simulink library "ParameterManager"  (R2025b)
settings: Solver=ode45  StartTime=0.0  StopTime=10.0  RelTol=1e-3  EnableMultiTasking=on
PreLoadFcn:
  | % Please do not Clear this line:
  | %damos=1;
undefined symbols (not defined in the file or in its folder): AD_DrvM_tSTATEIDX_E, u2, u3
libraries: CalibrationLib x21, simulink x10, $bdroot x2
settings Model: Creator=gaz2si  LastModifiedBy=JVE2ST
settings Model: ModifiedHistory=|
  | v7 15.10.2018
  | -Bus Signals removed
  | 
  | v6 07.03.2018
  | 
  | idq current swich in mot param 500us is changed, because of review. No functional changes, only layout.
  | 
  | v5 12.02.2018
  | 
  | Proc Ecu 500us is cahnged because of unit test. One More layer is added.
  | No Functional Changes.
  | 
  | ######################################################################
  | Model Version v4 - 17.08.2017 - ZYU8SI:
  | --------------------------------------------------------------------------------------
  | Developed for SW-Version: 320320_D0101
  | Used in customer projects: Plattform
  | Restrictions:
  | ---------------------------------------------------------------------------------------
  | Changed Interfaces:  - add I/O-Interfaces: fFamosReqd
  | --------------------------------------------------------------------------------------
  | Description:
  | - terminate ComWrp_Outp_iMaxChrgCurrent because no signal available from CAN
  | - set ComWrp_Outp_iChrgCurrDemand(maxDcCurrentOffset)=0. Variable needed for FAMOS
  | 
  | ######################################################################
  | Model Version v3 - 22.02.2017 - ZYU8SI:
  | --------------------------------------------------------------------------------------
  | Developed for SW-Version: latest
  | Used in customer projects: Daimler
  | Restrictions:
  | ---------------------------------------------------------------------------------------
  | Changed Interfaces:  none
  | --------------------------------------------------------------------------------------
  | Description:
  | - Split up model and included all functions as library
  | - from now on no functional development in this lib anymore
  | 
  | ######################################################################
  | 
  | 
  | SOO6SI v2 BMW Version:
  | - Interfaces IdcMin and IdcMax, ResBatteryCharge, ResBatteryDischarge are removed from the ComWrapper,
  |  and replaced by Damos Constants in the mask of the ECUParameter_5ms
  | 
  | ZSD2SI v1 BMW Version:
  | - Interfaces added: CustStMgr_OutP_sState_read
  | - Tq Gradient based on CustStMgr_OutP_sState_read (Torque Gradient has to be positive and in model it has to be set negative aus input)
  | - XCP value considered for Rising and falling Gradient
  | - ParameterManager/ProcEcu_500us/uPhaC_Srv_GetStrtNxtOutpWin set datatype from CSUINT32 to uint32
  | - Multiplikation of coefficients psi_d and psi_q with factor 10^-7
settings SolverCC: AlgebraicLoopSolver=TrustRegion
settings DataIOCC: LimitDataPoints=on  SaveFormat=Array  ReturnWorkspaceOutputs=off
settings OptimizationCC: LifeSpan=inf
settings DebuggingCC: SolverPrmCheckMsg=warning  UnconnectedInputMsg=warning  UnconnectedOutputMsg=warning  UnconnectedLineMsg=warning  AllowSymbolicDim=off  SFUnexpectedBacktrackingDiag=warning  SFNoUnconditionalDefaultTransitionDiag=warning  SFExecutionAtInitializationDiag=none  ArithmeticOperatorsInVariantConditions=warning
settings HardwareCC: ProdBitPerPointer=32.0  ProdBitPerSizeT=32.0  ProdBitPerPtrDiffT=32.0  ProdLargestAtomicFloat=None  ProdIntDivRoundTo=Undefined  ProdEndianess=Unspecified  ProdWordSize=32.0  ProdHWDeviceType=32-bit Generic
settings ModelReferenceCC: EnableRefExpFcnMdlSchedulingChecks=on  PropagateSignalLabelsOutOfModel=off
settings SFSimCC: SimUseLocalCustomCode=off  CustomCodeUndefinedFunction=UseInterfaceOnly
settings RTWCC: RTWUseLocalCustomCode=off  GPUComputeCapability=3.5
settings CodeAppCC: StateflowObjectComments=on
settings GRTTargetCC: TargetLangStandard=C89/C90 (ANSI)
settings ConfigComp: CovMetricSettings=dw  CovSaveCumulativeToWorkspaceVar=on  CovSaveSingleToWorkspaceVar=on  CovExternalEMLEnable=off  CovSFcnEnable=off

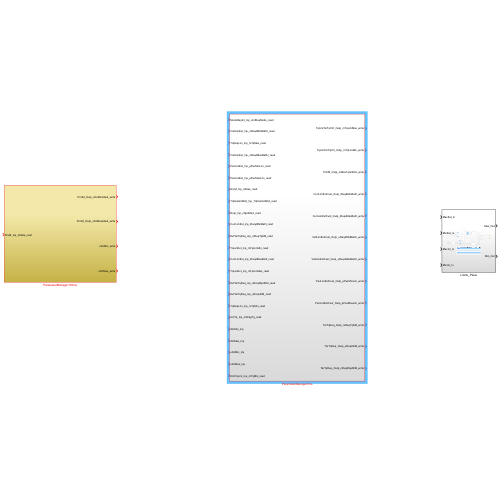
[thumbnail: Simulink's stored preview of the top-level diagram]
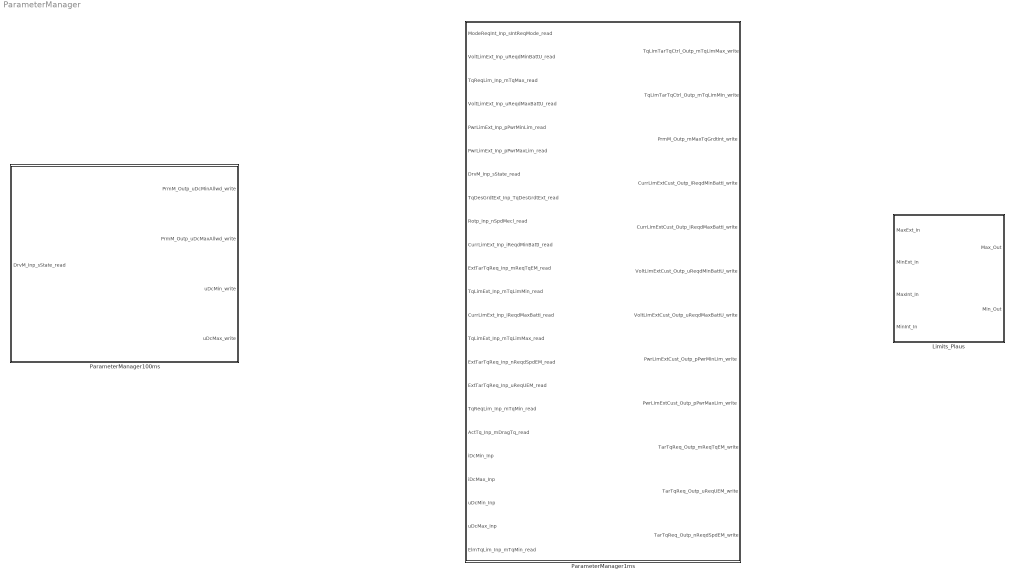
== system ParameterManager ==
  Limits_Plaus : Subsystem
  ParameterManager100ms : Subsystem
  ParameterManager1ms : Subsystem

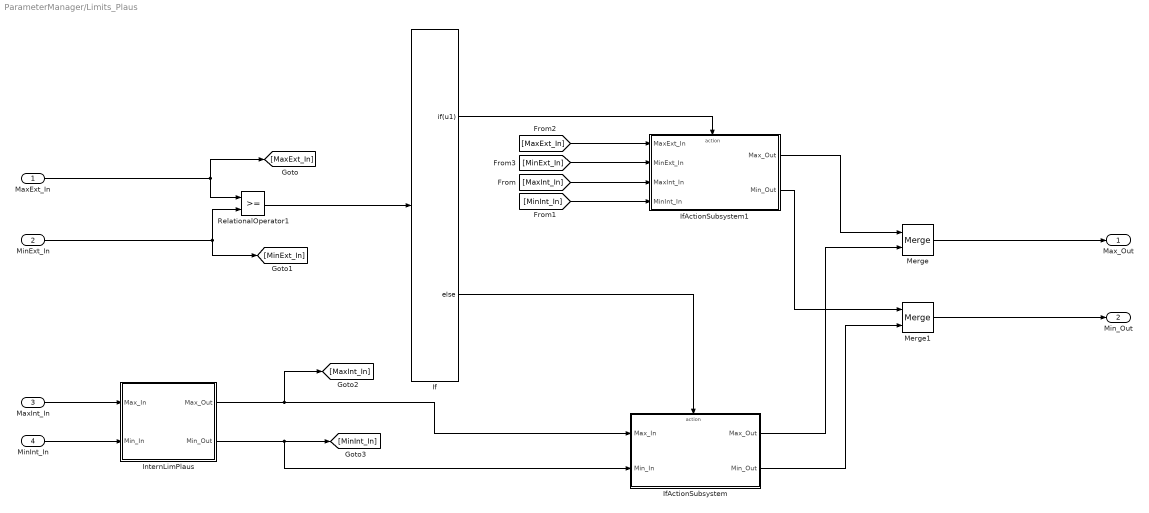
== system ParameterManager/Limits_Plaus ==
  MaxExt_In : Inport
  MinExt_In : Inport  Port=2
  MaxInt_In : Inport  Port=3
  MinInt_In : Inport  Port=4
  If : If  IfExpression=u1
  IfActionSubsystem : Subsystem  TreatAsAtomicUnit=on
  IfActionSubsystem1 : Subsystem  TreatAsAtomicUnit=on
  InternLimPlaus : Subsystem
  Merge : Merge
  Merge1 : Merge
  RelationalOperator1 : RelationalOperator  OutDataTypeStr=boolean  RndMeth=Simplest  InputSameDT=off
  Max_Out : Outport  VectorParamsAs1DForOutWhenUnconnected=off
  Min_Out : Outport  Port=2  VectorParamsAs1DForOutWhenUnconnected=off
  wires:
  If/1 -> IfActionSubsystem1/Action
  RelationalOperator1/1 -> If/1
  MinExt_In/1 -> [MinExt_In], RelationalOperator1/2
  MaxExt_In/1 -> [MaxExt_In], RelationalOperator1/1
  [MinInt_In] -> IfActionSubsystem1/4(MinInt_In)
  InternLimPlaus/2(Min_Out) -> IfActionSubsystem/2(Min_In), [MinInt_In]
  [MaxInt_In] -> IfActionSubsystem1/3(MaxInt_In)
  Merge/1 -> Max_Out/1
  [MaxExt_In] -> IfActionSubsystem1/1(MaxExt_In)
  [MinExt_In] -> IfActionSubsystem1/2(MinExt_In)
  If/2 -> IfActionSubsystem/Action
  InternLimPlaus/1(Max_Out) -> [MaxInt_In], IfActionSubsystem/1(Max_In)
  IfActionSubsystem1/2(Min_Out) -> Merge1/1
  IfActionSubsystem/1(Max_Out) -> Merge/2
  IfActionSubsystem1/1(Max_Out) -> Merge/1
  Merge1/1 -> Min_Out/1
  IfActionSubsystem/2(Min_Out) -> Merge1/2
  MaxInt_In/1 -> InternLimPlaus/1(Max_In)
  MinInt_In/1 -> InternLimPlaus/2(Min_In)

== system ParameterManager/ParameterManager100ms ==
  DrvM_Inp_sState_read : Inport
  ElectricalLimits : Subsystem
  SendingParameters : Subsystem
  PrmM_Outp_uDcMinAllwd_write : Outport  OutDataTypeStr=single  VectorParamsAs1DForOutWhenUnconnected=off
  PrmM_Outp_uDcMaxAllwd_write : Outport  Port=2  OutDataTypeStr=single  VectorParamsAs1DForOutWhenUnconnected=off
  uDcMin_write : Outport  Port=3  OutMin=24  OutMax=54  OutDataTypeStr=AD_PrmM_tUDCMINALLWD  PortDimensions=1  VectorParamsAs1DForOutWhenUnconnected=off
  uDcMax_write : Outport  Port=4  OutMin=24  OutMax=54  OutDataTypeStr=AD_PrmM_tUDCMAXALLWD  PortDimensions=1  VectorParamsAs1DForOutWhenUnconnected=off
  wires:
  DrvM_Inp_sState_read/1 -> ElectricalLimits/1(sState)
  ElectricalLimits/1(uDcMin_write) -> SendingParameters/1(uDcMin), uDcMin_write/1
  ElectricalLimits/2(uDcMax_write) -> SendingParameters/2(uDcMax), uDcMax_write/1
  SendingParameters/1(uDcMin_write) -> PrmM_Outp_uDcMinAllwd_write/1
  SendingParameters/2(uDcMax_write) -> PrmM_Outp_uDcMaxAllwd_write/1

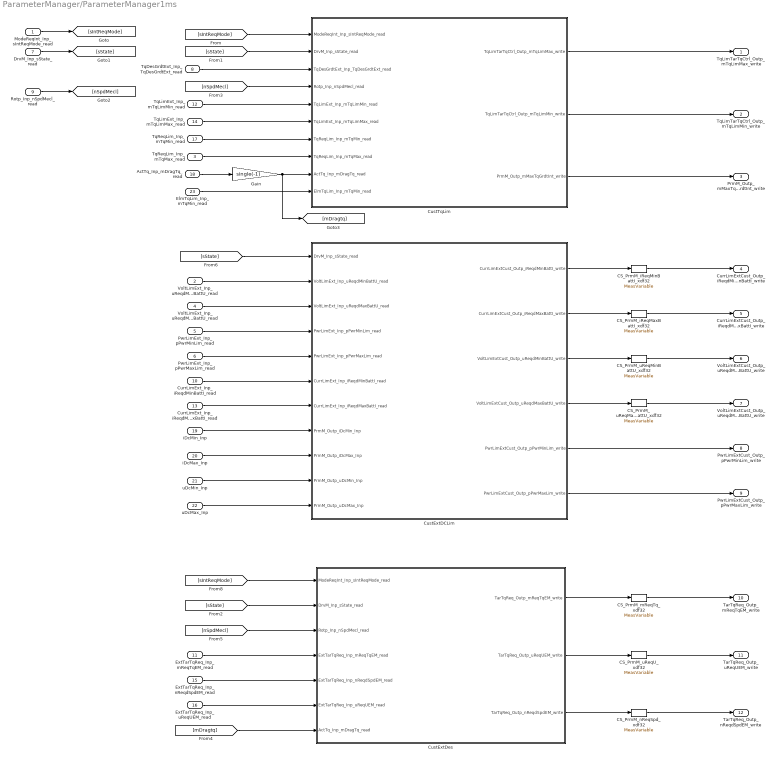
== system ParameterManager/ParameterManager1ms ==
  ModeReqInt_Inp_sIntReqMode_read : Inport
  VoltLimExt_Inp_uReqdMinBattU_read : Inport  Port=2
  TqReqLim_Inp_mTqMax_read : Inport  Port=3
  VoltLimExt_Inp_uReqdMaxBattU_read : Inport  Port=4
  PwrLimExt_Inp_pPwrMinLim_read : Inport  Port=5
  PwrLimExt_Inp_pPwrMaxLim_read : Inport  Port=6
  DrvM_Inp_sState_read : Inport  Port=7
  TqDesGrdtExt_Inp_TqDesGrdtExt_read : Inport  Port=8
  Rotp_Inp_nSpdMecl_read : Inport  Port=9
  CurrLimExt_Inp_iReqdMinBattI_read : Inport  Port=10
  ExtTarTqReq_Inp_mReqTqEM_read : Inport  Port=11
  TqLimExt_Inp_mTqLimMin_read : Inport  Port=12
  CurrLimExt_Inp_iReqdMaxBattI_read : Inport  Port=13
  TqLimExt_Inp_mTqLimMax_read : Inport  Port=14
  ExtTarTqReq_Inp_nReqdSpdEM_read : Inport  Port=15
  ExtTarTqReq_Inp_uReqUEM_read : Inport  Port=16
  TqReqLim_Inp_mTqMin_read : Inport  Port=17
  ActTq_Inp_mDragTq_read : Inport  Port=18
  iDcMin_Inp : Inport  Port=19
  iDcMax_Inp : Inport  Port=20
  uDcMin_Inp : Inport  Port=21
  uDcMax_Inp : Inport  Port=22
  ElmTqLim_Inp_mTqMin_read : Inport  Port=23
  CS_PrmM_iReqMaxBattI_xdf32 : CalibrationLib/MeasVariable  calSigName=CS_PrmM_iReqMaxBattI_xdf32  logSignal=on
      settings: AttributesFormatString=%<calSigName>  SourceProductName=SEG Calibration Lib
  CS_PrmM_iReqMinBattI_xdf32 : CalibrationLib/MeasVariable  calSigName=CS_PrmM_iReqMinBattI_xdf32  logSignal=on
      settings: AttributesFormatString=%<calSigName>  SourceProductName=SEG Calibration Lib
  CS_PrmM_mReqTq_xdf32 : CalibrationLib/MeasVariable  calSigName=CS_PrmM_mReqTq_xdf32  logSignal=on
      settings: AttributesFormatString=%<calSigName>  SourceProductName=SEG Calibration Lib
  CS_PrmM_nReqSpd_xdf32 : CalibrationLib/MeasVariable  calSigName=CS_PrmM_nReqSpd_xdf32  logSignal=on
      settings: AttributesFormatString=%<calSigName>  SourceProductName=SEG Calibration Lib
  CS_PrmM_uReqMaxBattU_xdf32 : CalibrationLib/MeasVariable  calSigName=CS_PrmM_uReqMaxBattU_xdf32  logSignal=on
      settings: AttributesFormatString=%<calSigName>  SourceProductName=SEG Calibration Lib
  CS_PrmM_uReqMinBattU_xdf32 : CalibrationLib/MeasVariable  calSigName=CS_PrmM_uReqMinBattU_xdf32  logSignal=on
      settings: AttributesFormatString=%<calSigName>  SourceProductName=SEG Calibration Lib
  CS_PrmM_uReqU_xdf32 : CalibrationLib/MeasVariable  calSigName=CS_PrmM_uReqU_xdf32  logSignal=on
      settings: AttributesFormatString=%<calSigName>  SourceProductName=SEG Calibration Lib
  CustExtDCLim : Subsystem
  CustExtDes : Subsystem
  CustTqLim : Subsystem
  Gain : Gain  Gain=single(-1)
  TqLimTarTqCtrl_Outp_mTqLimMax_write : Outport  VectorParamsAs1DForOutWhenUnconnected=off
      settings: EnsureOutportIsVirtual=on
  TqLimTarTqCtrl_Outp_mTqLimMin_write : Outport  Port=2  VectorParamsAs1DForOutWhenUnconnected=off
      settings: EnsureOutportIsVirtual=on
  PrmM_Outp_mMaxTqGrdtInt_write : Outport  Port=3  VectorParamsAs1DForOutWhenUnconnected=off
      settings: EnsureOutportIsVirtual=on
  CurrLimExtCust_Outp_iReqdMinBattI_write : Outport  Port=4  VectorParamsAs1DForOutWhenUnconnected=off
      settings: EnsureOutportIsVirtual=on
  CurrLimExtCust_Outp_iReqdMaxBattI_write : Outport  Port=5  VectorParamsAs1DForOutWhenUnconnected=off
      settings: EnsureOutportIsVirtual=on
  VoltLimExtCust_Outp_uReqdMinBattU_write : Outport  Port=6  VectorParamsAs1DForOutWhenUnconnected=off
      settings: EnsureOutportIsVirtual=on
  VoltLimExtCust_Outp_uReqdMaxBattU_write : Outport  Port=7  VectorParamsAs1DForOutWhenUnconnected=off
      settings: EnsureOutportIsVirtual=on
  PwrLimExtCust_Outp_pPwrMinLim_write : Outport  Port=8  VectorParamsAs1DForOutWhenUnconnected=off
      settings: EnsureOutportIsVirtual=on
  PwrLimExtCust_Outp_pPwrMaxLim_write : Outport  Port=9  VectorParamsAs1DForOutWhenUnconnected=off
      settings: EnsureOutportIsVirtual=on
  TarTqReq_Outp_mReqTqEM_write : Outport  Port=10  VectorParamsAs1DForOutWhenUnconnected=off
      settings: EnsureOutportIsVirtual=on
  TarTqReq_Outp_uReqUEM_write : Outport  Port=11  VectorParamsAs1DForOutWhenUnconnected=off
      settings: EnsureOutportIsVirtual=on
  TarTqReq_Outp_nReqdSpdEM_write : Outport  Port=12  VectorParamsAs1DForOutWhenUnconnected=off
      settings: EnsureOutportIsVirtual=on
  wires:
  Gain/1 -> [mDragtq], CustTqLim/9(ActTq_Inp_mDragTq_read)
  [mDragtq] -> CustExtDes/7(ActTq_Inp_mDragTq_read)
  ElmTqLim_Inp_mTqMin_read/1 -> CustTqLim/10(ElmTqLim_Inp_mTqMin_read)
  TqReqLim_Inp_mTqMax_read/1 -> CustTqLim/8(TqReqLim_Inp_mTqMax_read)
  VoltLimExt_Inp_uReqdMaxBattU_read/1 -> CustExtDCLim/3(VoltLimExt_Inp_uReqdMaxBattU_read)
  PwrLimExt_Inp_pPwrMinLim_read/1 -> CustExtDCLim/4(PwrLimExt_Inp_pPwrMinLim_read)
  PwrLimExt_Inp_pPwrMaxLim_read/1 -> CustExtDCLim/5(PwrLimExt_Inp_pPwrMaxLim_read)
  DrvM_Inp_sState_read/1 -> [sState]
  TqDesGrdtExt_Inp_TqDesGrdtExt_read/1 -> CustTqLim/3(TqDesGrdtExt_Inp_TqDesGrdtExt_read)
  Rotp_Inp_nSpdMecl_read/1 -> [nSpdMecl]
  CurrLimExt_Inp_iReqdMinBattI_read/1 -> CustExtDCLim/6(CurrLimExt_Inp_iReqdMinBattI_read)
  ExtTarTqReq_Inp_mReqTqEM_read/1 -> CustExtDes/4(ExtTarTqReq_Inp_mReqTqEM_read)
  TqLimExt_Inp_mTqLimMin_read/1 -> CustTqLim/5(TqLimExt_Inp_mTqLimMin_read)
  CurrLimExt_Inp_iReqdMaxBattI_read/1 -> CustExtDCLim/7(CurrLimExt_Inp_iReqdMaxBattI_read)
  TqLimExt_Inp_mTqLimMax_read/1 -> CustTqLim/6(TqLimExt_Inp_mTqLimMax_read)
  ExtTarTqReq_Inp_nReqdSpdEM_read/1 -> CustExtDes/5(ExtTarTqReq_Inp_nReqdSpdEM_read)
  ExtTarTqReq_Inp_uReqUEM_read/1 -> CustExtDes/6(ExtTarTqReq_Inp_uReqUEM_read)
  ActTq_Inp_mDragTq_read/1 -> Gain/1
  CustExtDCLim/1(CurrLimExtCust_Outp_iReqdMinBattI_write) -> CS_PrmM_iReqMinBattI_xdf32/1
  CustExtDCLim/2(CurrLimExtCust_Outp_iReqdMaxBattI_write) -> CS_PrmM_iReqMaxBattI_xdf32/1
  CustExtDCLim/3(VoltLimExtCust_Outp_uReqdMinBattU_write) -> CS_PrmM_uReqMinBattU_xdf32/1
  CustExtDCLim/4(VoltLimExtCust_Outp_uReqdMaxBattU_write) -> CS_PrmM_uReqMaxBattU_xdf32/1
  CustExtDCLim/5(PwrLimExtCust_Outp_pPwrMinLim_write) -> PwrLimExtCust_Outp_pPwrMinLim_write/1
  CustExtDCLim/6(PwrLimExtCust_Outp_pPwrMaxLim_write) -> PwrLimExtCust_Outp_pPwrMaxLim_write/1
  CustExtDes/1(TarTqReq_Outp_mReqTqEM_write) -> CS_PrmM_mReqTq_xdf32/1
  CustExtDes/2(TarTqReq_Outp_uReqUEM_write) -> CS_PrmM_uReqU_xdf32/1
  CustExtDes/3(TarTqReq_Outp_nReqdSpdEM_write) -> CS_PrmM_nReqSpd_xdf32/1
  iDcMin_Inp/1 -> CustExtDCLim/8(PrmM_Outp_iDcMin_Inp)
  iDcMax_Inp/1 -> CustExtDCLim/9(PrmM_Outp_iDcMax_Inp)
  uDcMin_Inp/1 -> CustExtDCLim/10(PrmM_Outp_uDcMin_Inp)
  uDcMax_Inp/1 -> CustExtDCLim/11(PrmM_Outp_uDcMax_Inp)
  ModeReqInt_Inp_sIntReqMode_read/1 -> [sIntReqMode]
  [sIntReqMode] -> CustTqLim/1(ModeReqInt_Inp_sIntReqMode_read)
  [sIntReqMode] -> CustExtDes/1(ModeReqInt_Inp_sIntReqMode_read)
  [sState] -> CustTqLim/2(DrvM_Inp_sState_read)
  [sState] -> CustExtDes/2(DrvM_Inp_sState_read)
  TqReqLim_Inp_mTqMin_read/1 -> CustTqLim/7(TqReqLim_Inp_mTqMin_read)
  [nSpdMecl] -> CustTqLim/4(Rotp_Inp_nSpdMecl_read)
  VoltLimExt_Inp_uReqdMinBattU_read/1 -> CustExtDCLim/2(VoltLimExt_Inp_uReqdMinBattU_read)
  [nSpdMecl] -> CustExtDes/3(Rotp_Inp_nSpdMecl_read)
  CustTqLim/1(TqLimTarTqCtrl_Outp_mTqLimMax_write) -> TqLimTarTqCtrl_Outp_mTqLimMax_write/1
  CustTqLim/2(TqLimTarTqCtrl_Outp_mTqLimMin_write) -> TqLimTarTqCtrl_Outp_mTqLimMin_write/1
  CS_PrmM_iReqMinBattI_xdf32/1 -> CurrLimExtCust_Outp_iReqdMinBattI_write/1
  CS_PrmM_iReqMaxBattI_xdf32/1 -> CurrLimExtCust_Outp_iReqdMaxBattI_write/1
  CS_PrmM_uReqMinBattU_xdf32/1 -> VoltLimExtCust_Outp_uReqdMinBattU_write/1
  CS_PrmM_mReqTq_xdf32/1 -> TarTqReq_Outp_mReqTqEM_write/1
  CS_PrmM_uReqU_xdf32/1 -> TarTqReq_Outp_uReqUEM_write/1
  CS_PrmM_nReqSpd_xdf32/1 -> TarTqReq_Outp_nReqdSpdEM_write/1
  CS_PrmM_uReqMaxBattU_xdf32/1 -> VoltLimExtCust_Outp_uReqdMaxBattU_write/1
  CustTqLim/3(PrmM_Outp_mMaxTqGrdtInt_write) -> PrmM_Outp_mMaxTqGrdtInt_write/1
  [sState] -> CustExtDCLim/1(DrvM_Inp_sState_read)

== system ParameterManager/Limits_Plaus/IfActionSubsystem ==
  Max_In : Inport
  Min_In : Inport  Port=2
  ActionPort : ActionPort
  Max_Out : Outport  VectorParamsAs1DForOutWhenUnconnected=off
  Min_Out : Outport  Port=2  VectorParamsAs1DForOutWhenUnconnected=off
  wires:
  Max_In/1 -> Max_Out/1
  Min_In/1 -> Min_Out/1

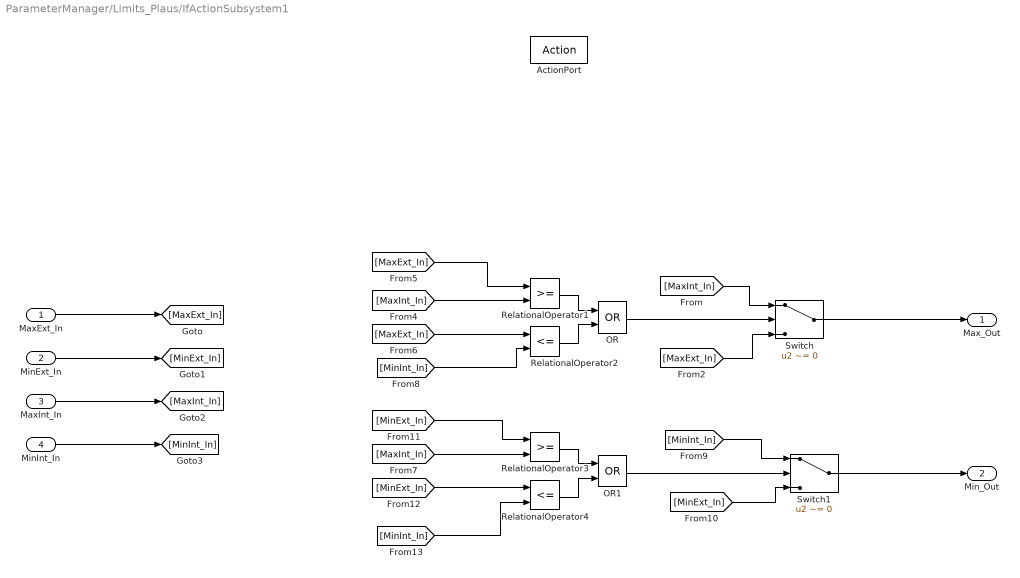
== system ParameterManager/Limits_Plaus/IfActionSubsystem1 ==
  MaxExt_In : Inport
  MinExt_In : Inport  Port=2
  MaxInt_In : Inport  Port=3
  MinInt_In : Inport  Port=4
  ActionPort : ActionPort  ActionPortLabel=if { }
  OR : Logic  Operator=OR  AllPortsSameDT=off  OutDataTypeStr=boolean
  OR1 : Logic  Operator=OR  AllPortsSameDT=off  OutDataTypeStr=boolean
  RelationalOperator1 : RelationalOperator  OutDataTypeStr=boolean  RndMeth=Simplest  InputSameDT=off
  RelationalOperator2 : RelationalOperator  Operator=<=  OutDataTypeStr=boolean  RndMeth=Simplest  InputSameDT=off
  RelationalOperator3 : RelationalOperator  OutDataTypeStr=boolean  RndMeth=Simplest  InputSameDT=off
  RelationalOperator4 : RelationalOperator  Operator=<=  OutDataTypeStr=boolean  RndMeth=Simplest  InputSameDT=off
  Switch : Switch  Criteria=u2 ~= 0  SaturateOnIntegerOverflow=off  InputSameDT=off
  Switch1 : Switch  Criteria=u2 ~= 0  SaturateOnIntegerOverflow=off  InputSameDT=off
  Max_Out : Outport  VectorParamsAs1DForOutWhenUnconnected=off
  Min_Out : Outport  Port=2  VectorParamsAs1DForOutWhenUnconnected=off
  wires:
  Switch1/1 -> Min_Out/1
  Switch/1 -> Max_Out/1
  MaxExt_In/1 -> [MaxExt_In]
  MaxInt_In/1 -> [MaxInt_In]
  MinInt_In/1 -> [MinInt_In]
  RelationalOperator1/1 -> OR/1
  RelationalOperator2/1 -> OR/2
  OR/1 -> Switch/2
  RelationalOperator4/1 -> OR1/2
  RelationalOperator3/1 -> OR1/1
  OR1/1 -> Switch1/2
  MinExt_In/1 -> [MinExt_In]
  [MaxExt_In] -> Switch/3
  [MaxInt_In] -> Switch/1
  [MaxInt_In] -> RelationalOperator1/2
  [MaxExt_In] -> RelationalOperator1/1
  [MaxExt_In] -> RelationalOperator2/1
  [MaxInt_In] -> RelationalOperator3/2
  [MinInt_In] -> RelationalOperator2/2
  [MinInt_In] -> Switch1/1
  [MinExt_In] -> Switch1/3
  [MinExt_In] -> RelationalOperator3/1
  [MinExt_In] -> RelationalOperator4/1
  [MinInt_In] -> RelationalOperator4/2

== system ParameterManager/Limits_Plaus/InternLimPlaus ==
  Max_In : Inport
  Min_In : Inport  Port=2
  RelationalOperator1 : RelationalOperator  OutDataTypeStr=boolean  RndMeth=Simplest  InputSameDT=off
  Switch : Switch  Criteria=u2 ~= 0  SaturateOnIntegerOverflow=off  InputSameDT=off
  Switch1 : Switch  Criteria=u2 ~= 0  SaturateOnIntegerOverflow=off  InputSameDT=off
  Max_Out : Outport  VectorParamsAs1DForOutWhenUnconnected=off
  Min_Out : Outport  Port=2  VectorParamsAs1DForOutWhenUnconnected=off
  wires:
  RelationalOperator1/1 -> Switch1/2, Switch/2
  Max_In/1 -> Switch1/3, Switch/1, RelationalOperator1/1
  Switch/1 -> Max_Out/1
  Switch1/1 -> Min_Out/1
  Min_In/1 -> RelationalOperator1/2, Switch/3, Switch1/1

== system ParameterManager/ParameterManager100ms/ElectricalLimits ==
  sState : Inport
  BatterylessOperation : Subsystem  TreatAsAtomicUnit=on
  CompareToConstant : simulink/Logic and Bit Operations/Compare To Constant  relop===  const=AD_DrvM_tSTATEIDX_E.CS_DrvM_STATE_BattDiscnctd  OutDataTypeStr=boolean
  CompareToConstant1 : simulink/Logic and Bit Operations/Compare To Constant  relop===  const=AD_DrvM_tSTATEIDX_E.CS_DrvM_STATE_Volt  OutDataTypeStr=boolean
  If : If  NumInputs=2  IfExpression=u1  ElseIfExpressions=u2
  Merge : Merge  Inputs=3
  Merge1 : Merge  Inputs=3
  Other : Subsystem  TreatAsAtomicUnit=on
  VoltageMode : Subsystem  TreatAsAtomicUnit=on
  uDcMin_write : Outport  OutMin=20  OutMax=65  OutDataTypeStr=AD_PrmM_tUDCMINALLWD  PortDimensions=1  VectorParamsAs1DForOutWhenUnconnected=off
  uDcMax_write : Outport  Port=2  OutMin=20  OutMax=65  OutDataTypeStr=AD_PrmM_tUDCMAXALLWD  PortDimensions=1  VectorParamsAs1DForOutWhenUnconnected=off
  wires:
  Other/1(uUmin) -> Merge/3
  CompareToConstant/1 -> If/1
  VoltageMode/2(uUmax) -> Merge1/2
  CompareToConstant1/1 -> If/2
  If/1 -> BatterylessOperation/Action
  sState/1 -> CompareToConstant1/1, CompareToConstant/1
  Merge1/1 -> uDcMax_write/1
  VoltageMode/1(uUmin) -> Merge/2
  If/2 -> VoltageMode/Action
  If/3 -> Other/Action
  BatterylessOperation/1(uUmin) -> Merge/1
  BatterylessOperation/2(uUmax) -> Merge1/1
  Other/2(uUmax) -> Merge1/3
  Merge/1 -> uDcMin_write/1

== system ParameterManager/ParameterManager100ms/SendingParameters ==
  uDcMin : Inport
  uDcMax : Inport  Port=2
  uDcMin_write : Outport  OutMin=20  OutMax=65  OutDataTypeStr=AD_PrmM_tUDCMINALLWD  PortDimensions=1  VectorParamsAs1DForOutWhenUnconnected=off
  uDcMax_write : Outport  Port=2  OutMin=20  OutMax=65  OutDataTypeStr=AD_PrmM_tUDCMAXALLWD  PortDimensions=1  VectorParamsAs1DForOutWhenUnconnected=off
  wires:
  uDcMin/1 -> uDcMin_write/1
  uDcMax/1 -> uDcMax_write/1

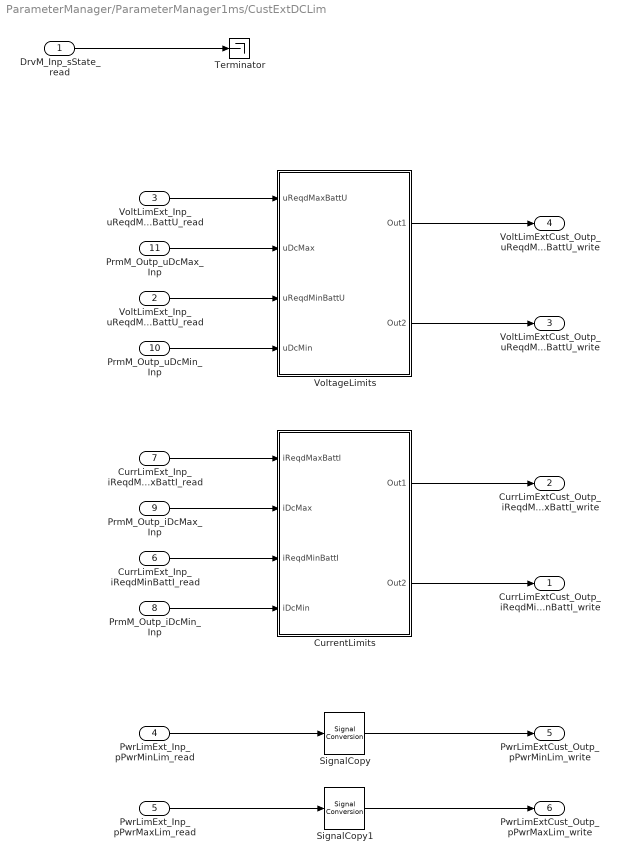
== system ParameterManager/ParameterManager1ms/CustExtDCLim ==
  DrvM_Inp_sState_read : Inport
  VoltLimExt_Inp_uReqdMinBattU_read : Inport  Port=2
  VoltLimExt_Inp_uReqdMaxBattU_read : Inport  Port=3
  PwrLimExt_Inp_pPwrMinLim_read : Inport  Port=4
  PwrLimExt_Inp_pPwrMaxLim_read : Inport  Port=5
  CurrLimExt_Inp_iReqdMinBattI_read : Inport  Port=6
  CurrLimExt_Inp_iReqdMaxBattI_read : Inport  Port=7
  PrmM_Outp_iDcMin_Inp : Inport  Port=8
  PrmM_Outp_iDcMax_Inp : Inport  Port=9
  PrmM_Outp_uDcMin_Inp : Inport  Port=10
  PrmM_Outp_uDcMax_Inp : Inport  Port=11
  CurrentLimits : Subsystem
  SignalCopy : SignalConversion  OverrideOpt=off
  SignalCopy1 : SignalConversion  OverrideOpt=off
  Terminator : Terminator
  VoltageLimits : Subsystem
  CurrLimExtCust_Outp_iReqdMinBattI_write : Outport  VectorParamsAs1DForOutWhenUnconnected=off
      settings: EnsureOutportIsVirtual=on
  CurrLimExtCust_Outp_iReqdMaxBattI_write : Outport  Port=2  VectorParamsAs1DForOutWhenUnconnected=off
      settings: EnsureOutportIsVirtual=on
  VoltLimExtCust_Outp_uReqdMinBattU_write : Outport  Port=3  VectorParamsAs1DForOutWhenUnconnected=off
      settings: EnsureOutportIsVirtual=on
  VoltLimExtCust_Outp_uReqdMaxBattU_write : Outport  Port=4  VectorParamsAs1DForOutWhenUnconnected=off
      settings: EnsureOutportIsVirtual=on
  PwrLimExtCust_Outp_pPwrMinLim_write : Outport  Port=5  VectorParamsAs1DForOutWhenUnconnected=off
      settings: EnsureOutportIsVirtual=on
  PwrLimExtCust_Outp_pPwrMaxLim_write : Outport  Port=6  VectorParamsAs1DForOutWhenUnconnected=off
      settings: EnsureOutportIsVirtual=on
  wires:
  VoltLimExt_Inp_uReqdMaxBattU_read/1 -> VoltageLimits/1(uReqdMaxBattU)
  PrmM_Outp_uDcMax_Inp/1 -> VoltageLimits/2(uDcMax)
  VoltLimExt_Inp_uReqdMinBattU_read/1 -> VoltageLimits/3(uReqdMinBattU)
  PrmM_Outp_uDcMin_Inp/1 -> VoltageLimits/4(uDcMin)
  VoltageLimits/1(Out1) -> VoltLimExtCust_Outp_uReqdMaxBattU_write/1
  VoltageLimits/2(Out2) -> VoltLimExtCust_Outp_uReqdMinBattU_write/1
  CurrentLimits/2(Out2) -> CurrLimExtCust_Outp_iReqdMinBattI_write/1
  CurrentLimits/1(Out1) -> CurrLimExtCust_Outp_iReqdMaxBattI_write/1
  CurrLimExt_Inp_iReqdMaxBattI_read/1 -> CurrentLimits/1(iReqdMaxBattI)
  PrmM_Outp_iDcMax_Inp/1 -> CurrentLimits/2(iDcMax)
  PrmM_Outp_iDcMin_Inp/1 -> CurrentLimits/4(iDcMin)
  CurrLimExt_Inp_iReqdMinBattI_read/1 -> CurrentLimits/3(iReqdMinBattI)
  PwrLimExt_Inp_pPwrMaxLim_read/1 -> SignalCopy1/1
  SignalCopy/1 -> PwrLimExtCust_Outp_pPwrMinLim_write/1
  SignalCopy1/1 -> PwrLimExtCust_Outp_pPwrMaxLim_write/1
  PwrLimExt_Inp_pPwrMinLim_read/1 -> SignalCopy/1
  DrvM_Inp_sState_read/1 -> Terminator/1

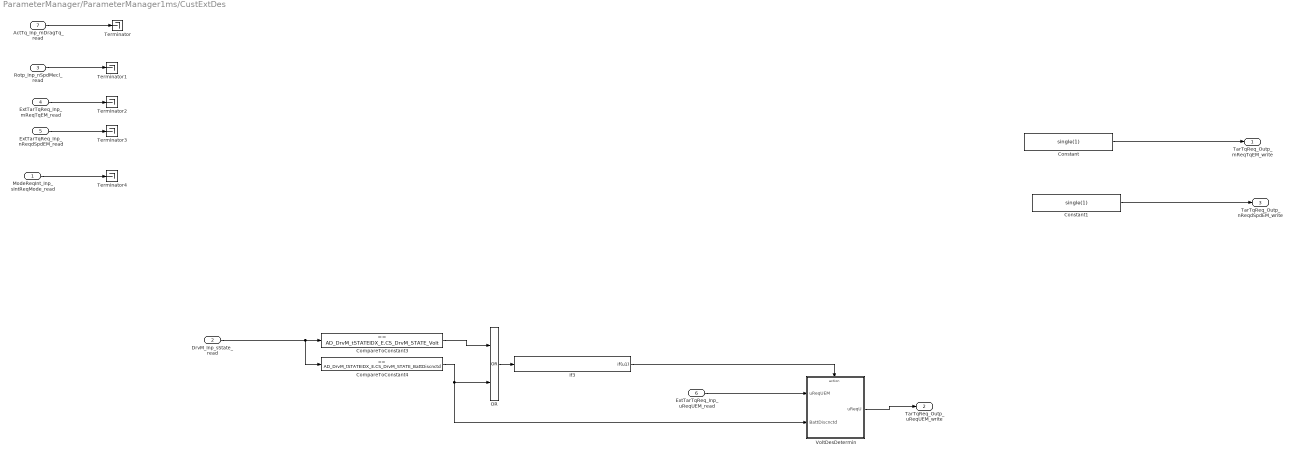
== system ParameterManager/ParameterManager1ms/CustExtDes ==
  ModeReqInt_Inp_sIntReqMode_read : Inport
  DrvM_Inp_sState_read : Inport  Port=2
  Rotp_Inp_nSpdMecl_read : Inport  Port=3
  ExtTarTqReq_Inp_mReqTqEM_read : Inport  Port=4
  ExtTarTqReq_Inp_nReqdSpdEM_read : Inport  Port=5
  ExtTarTqReq_Inp_uReqUEM_read : Inport  Port=6
  ActTq_Inp_mDragTq_read : Inport  Port=7
  CompareToConstant3 : simulink/Logic and Bit Operations/Compare To Constant  relop===  const=AD_DrvM_tSTATEIDX_E.CS_DrvM_STATE_Volt  OutDataTypeStr=boolean
  CompareToConstant4 : simulink/Logic and Bit Operations/Compare To Constant  relop===  const=AD_DrvM_tSTATEIDX_E.CS_DrvM_STATE_BattDiscnctd  OutDataTypeStr=boolean
  Constant : Constant  Value=single(1)
  Constant1 : Constant  Value=single(1)
  If3 : If  IfExpression=u1  ShowElse=off
  OR : Logic  Operator=OR  AllPortsSameDT=off  OutDataTypeStr=boolean
  Terminator{,1..4} (5 alike) : Terminator
  VoltDesDetermin : Subsystem  TreatAsAtomicUnit=on
  TarTqReq_Outp_mReqTqEM_write : Outport  VectorParamsAs1DForOutWhenUnconnected=off
      settings: EnsureOutportIsVirtual=on
  TarTqReq_Outp_uReqUEM_write : Outport  Port=2  VectorParamsAs1DForOutWhenUnconnected=off
      settings: EnsureOutportIsVirtual=on
  TarTqReq_Outp_nReqdSpdEM_write : Outport  Port=3  VectorParamsAs1DForOutWhenUnconnected=off
      settings: EnsureOutportIsVirtual=on
  wires:
  ExtTarTqReq_Inp_uReqUEM_read/1 -> VoltDesDetermin/1(uReqUEM)
  Constant1/1 -> TarTqReq_Outp_nReqdSpdEM_write/1
  DrvM_Inp_sState_read/1 -> CompareToConstant3/1, CompareToConstant4/1
  OR/1 -> If3/1
  CompareToConstant3/1 -> OR/1
  CompareToConstant4/1 -> VoltDesDetermin/2(BattDiscnctd), OR/2
  VoltDesDetermin/1(uReqU) -> TarTqReq_Outp_uReqUEM_write/1
  If3/1 -> VoltDesDetermin/Action
  ActTq_Inp_mDragTq_read/1 -> Terminator/1
  Rotp_Inp_nSpdMecl_read/1 -> Terminator1/1
  ExtTarTqReq_Inp_nReqdSpdEM_read/1 -> Terminator3/1
  ExtTarTqReq_Inp_mReqTqEM_read/1 -> Terminator2/1
  ModeReqInt_Inp_sIntReqMode_read/1 -> Terminator4/1
  Constant/1 -> TarTqReq_Outp_mReqTqEM_write/1

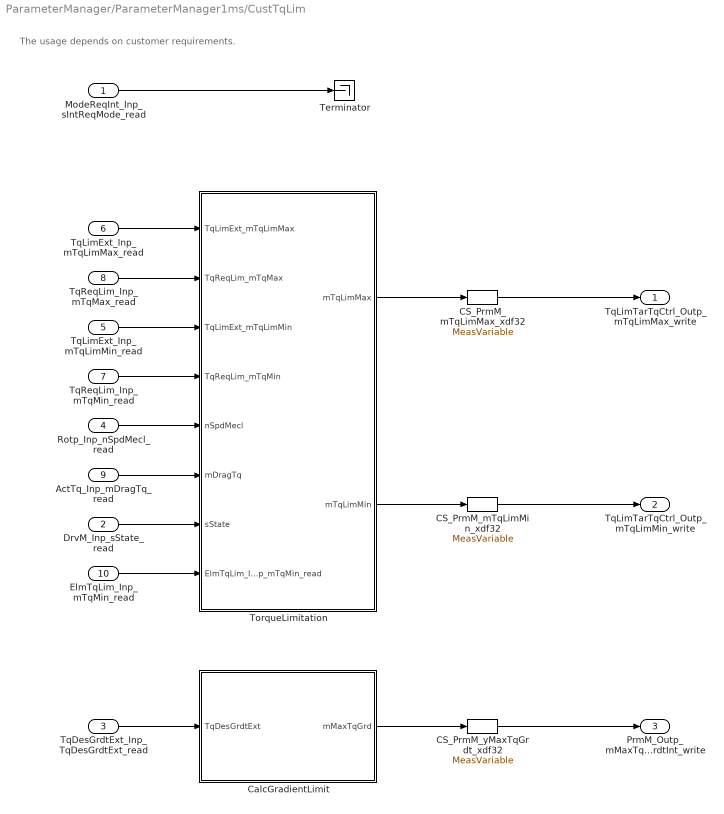
== system ParameterManager/ParameterManager1ms/CustTqLim ==
  note: The usage depends on customer requirements.
  ModeReqInt_Inp_sIntReqMode_read : Inport
  DrvM_Inp_sState_read : Inport  Port=2
  TqDesGrdtExt_Inp_TqDesGrdtExt_read : Inport  Port=3
  Rotp_Inp_nSpdMecl_read : Inport  Port=4
  TqLimExt_Inp_mTqLimMin_read : Inport  Port=5
  TqLimExt_Inp_mTqLimMax_read : Inport  Port=6
  TqReqLim_Inp_mTqMin_read : Inport  Port=7
  TqReqLim_Inp_mTqMax_read : Inport  Port=8
  ActTq_Inp_mDragTq_read : Inport  Port=9
  ElmTqLim_Inp_mTqMin_read : Inport  Port=10
  CS_PrmM_mTqLimMax_xdf32 : CalibrationLib/MeasVariable  calSigName=CS_PrmM_mTqLimMax_xdf32  logSignal=on
      settings: AttributesFormatString=%<calSigName>  SourceProductName=SEG Calibration Lib
  CS_PrmM_mTqLimMin_xdf32 : CalibrationLib/MeasVariable  calSigName=CS_PrmM_mTqLimMin_xdf32  logSignal=on
      settings: AttributesFormatString=%<calSigName>  SourceProductName=SEG Calibration Lib
  CS_PrmM_yMaxTqGrdt_xdf32 : CalibrationLib/MeasVariable  calSigName=CS_PrmM_yMaxTqGrdt_xdf32  logSignal=on
      settings: AttributesFormatString=%<calSigName>  SourceProductName=SEG Calibration Lib
  CalcGradientLimit : Subsystem
  Terminator : Terminator
  TorqueLimitation : Subsystem
  TqLimTarTqCtrl_Outp_mTqLimMax_write : Outport  VectorParamsAs1DForOutWhenUnconnected=off
      settings: EnsureOutportIsVirtual=on
  TqLimTarTqCtrl_Outp_mTqLimMin_write : Outport  Port=2  VectorParamsAs1DForOutWhenUnconnected=off
      settings: EnsureOutportIsVirtual=on
  PrmM_Outp_mMaxTqGrdtInt_write : Outport  Port=3  VectorParamsAs1DForOutWhenUnconnected=off
      settings: EnsureOutportIsVirtual=on
  wires:
  ElmTqLim_Inp_mTqMin_read/1 -> TorqueLimitation/8(ElmTqLim_Inp_mTqMin_read)
  ModeReqInt_Inp_sIntReqMode_read/1 -> Terminator/1
  TorqueLimitation/1(mTqLimMax) -> CS_PrmM_mTqLimMax_xdf32/1
  TqDesGrdtExt_Inp_TqDesGrdtExt_read/1 -> CalcGradientLimit/1(TqDesGrdtExt)
  CalcGradientLimit/1(mMaxTqGrd) -> CS_PrmM_yMaxTqGrdt_xdf32/1
  TqLimExt_Inp_mTqLimMax_read/1 -> TorqueLimitation/1(TqLimExt_mTqLimMax)
  TqReqLim_Inp_mTqMax_read/1 -> TorqueLimitation/2(TqReqLim_mTqMax)
  TqLimExt_Inp_mTqLimMin_read/1 -> TorqueLimitation/3(TqLimExt_mTqLimMin)
  TqReqLim_Inp_mTqMin_read/1 -> TorqueLimitation/4(TqReqLim_mTqMin)
  Rotp_Inp_nSpdMecl_read/1 -> TorqueLimitation/5(nSpdMecl)
  ActTq_Inp_mDragTq_read/1 -> TorqueLimitation/6(mDragTq)
  DrvM_Inp_sState_read/1 -> TorqueLimitation/7(sState)
  TorqueLimitation/2(mTqLimMin) -> CS_PrmM_mTqLimMin_xdf32/1
  CS_PrmM_mTqLimMax_xdf32/1 -> TqLimTarTqCtrl_Outp_mTqLimMax_write/1
  CS_PrmM_mTqLimMin_xdf32/1 -> TqLimTarTqCtrl_Outp_mTqLimMin_write/1
  CS_PrmM_yMaxTqGrdt_xdf32/1 -> PrmM_Outp_mMaxTqGrdtInt_write/1

== system ParameterManager/ParameterManager100ms/ElectricalLimits/BatterylessOperation ==
  ActionPort : ActionPort  ActionPortLabel=if { }
  CS_PrmM_uDcMaxBattLess_XDF32 : CalibrationLib/Parameter  calParamName=CS_PrmM_uDcMaxBattLess_XDF32
      settings: AttributesFormatString=%<calParamName>  SourceProductName=SEG Calibration Lib
  CS_PrmM_uDcMinBattLess_XDF32 : CalibrationLib/Parameter  calParamName=CS_PrmM_uDcMinBattLess_XDF32
      settings: AttributesFormatString=%<calParamName>  SourceProductName=SEG Calibration Lib
  uUmin : Outport  VectorParamsAs1DForOutWhenUnconnected=off
  uUmax : Outport  Port=2  VectorParamsAs1DForOutWhenUnconnected=off
  wires:
  CS_PrmM_uDcMaxBattLess_XDF32/1 -> uUmax/1
  CS_PrmM_uDcMinBattLess_XDF32/1 -> uUmin/1

== system ParameterManager/ParameterManager100ms/ElectricalLimits/Other ==
  ActionPort : ActionPort  ActionPortLabel=else { }
  CS_PrmM_uDcMaxOtherM_XDF32 : CalibrationLib/Parameter  calParamName=CS_PrmM_uDcMaxOtherM_XDF32
      settings: AttributesFormatString=%<calParamName>  SourceProductName=SEG Calibration Lib
  CS_PrmM_uDcMinOtherM_XDF32 : CalibrationLib/Parameter  calParamName=CS_PrmM_uDcMinOtherM_XDF32
      settings: AttributesFormatString=%<calParamName>  SourceProductName=SEG Calibration Lib
  uUmin : Outport  VectorParamsAs1DForOutWhenUnconnected=off
  uUmax : Outport  Port=2  VectorParamsAs1DForOutWhenUnconnected=off
  wires:
  CS_PrmM_uDcMinOtherM_XDF32/1 -> uUmin/1
  CS_PrmM_uDcMaxOtherM_XDF32/1 -> uUmax/1

== system ParameterManager/ParameterManager100ms/ElectricalLimits/VoltageMode ==
  ActionPort : ActionPort  ActionPortLabel=elseif { }
  CS_PrmM_uDcMaxVoltMode_XDF32 : CalibrationLib/Parameter  calParamName=CS_PrmM_uDcMaxVoltMode_XDF32
      settings: AttributesFormatString=%<calParamName>  SourceProductName=SEG Calibration Lib
  CS_PrmM_uDcMinVoltMode_XDF32 : CalibrationLib/Parameter  calParamName=CS_PrmM_uDcMinVoltMode_XDF32
      settings: AttributesFormatString=%<calParamName>  SourceProductName=SEG Calibration Lib
  uUmin : Outport  VectorParamsAs1DForOutWhenUnconnected=off
  uUmax : Outport  Port=2  VectorParamsAs1DForOutWhenUnconnected=off
  wires:
  CS_PrmM_uDcMaxVoltMode_XDF32/1 -> uUmax/1
  CS_PrmM_uDcMinVoltMode_XDF32/1 -> uUmin/1

== system ParameterManager/ParameterManager1ms/CustExtDCLim/CurrentLimits ==
  iReqdMaxBattI : Inport
  iDcMax : Inport  Port=2
  iReqdMinBattI : Inport  Port=3
  iDcMin : Inport  Port=4
  Limits_Plaus : $bdroot/Limits_Plaus  SystemSampleTime=-1  VariantActivationTime=update diagram  EmptyChoice=off  PassThrough=off  PassThroughVariantControl=(default)  EmptyChoiceVariantControl=(default)  AllowFlexibleInterface=on  Latency=0  AutoFrameSizeCalculation=off
  Out1 : Outport  VectorParamsAs1DForOutWhenUnconnected=off
  Out2 : Outport  Port=2  VectorParamsAs1DForOutWhenUnconnected=off
  wires:
  Limits_Plaus/1 -> Out1/1
  Limits_Plaus/2 -> Out2/1
  iReqdMaxBattI/1 -> Limits_Plaus/1
  iDcMax/1 -> Limits_Plaus/3
  iReqdMinBattI/1 -> Limits_Plaus/2
  iDcMin/1 -> Limits_Plaus/4

== system ParameterManager/ParameterManager1ms/CustExtDCLim/VoltageLimits ==
  uReqdMaxBattU : Inport
  uDcMax : Inport  Port=2
  uReqdMinBattU : Inport  Port=3
  uDcMin : Inport  Port=4
  Limits_Plaus : $bdroot/Limits_Plaus  SystemSampleTime=-1  VariantActivationTime=update diagram  EmptyChoice=off  PassThrough=off  PassThroughVariantControl=(default)  EmptyChoiceVariantControl=(default)  AllowFlexibleInterface=on  Latency=0  AutoFrameSizeCalculation=off
  Out1 : Outport  VectorParamsAs1DForOutWhenUnconnected=off
  Out2 : Outport  Port=2  VectorParamsAs1DForOutWhenUnconnected=off
  wires:
  Limits_Plaus/2 -> Out2/1
  Limits_Plaus/1 -> Out1/1
  uReqdMaxBattU/1 -> Limits_Plaus/1
  uReqdMinBattU/1 -> Limits_Plaus/2
  uDcMax/1 -> Limits_Plaus/3
  uDcMin/1 -> Limits_Plaus/4

== system ParameterManager/ParameterManager1ms/CustExtDes/VoltDesDetermin ==
  uReqUEM : Inport
  BattDiscnctd : Inport  Port=2
  ActionPort : ActionPort
  Saturation : Saturate  UpperLimit=single(54.5)  LowerLimit=single(24)
      settings: AttributesFormatString=|
      | UpperLim: %<UpperLimit>
      | LowerLim: %<LowerLimit>
  Switch1 : Switch  Criteria=u2 ~= 0  SaturateOnIntegerOverflow=off  InputSameDT=off
  uReqU : Outport  VectorParamsAs1DForOutWhenUnconnected=off
  wires:
  Switch1/1 -> uReqU/1
  BattDiscnctd/1 -> Switch1/2
  Saturation/1 -> Switch1/1
  uReqUEM/1 -> Switch1/3, Saturation/1

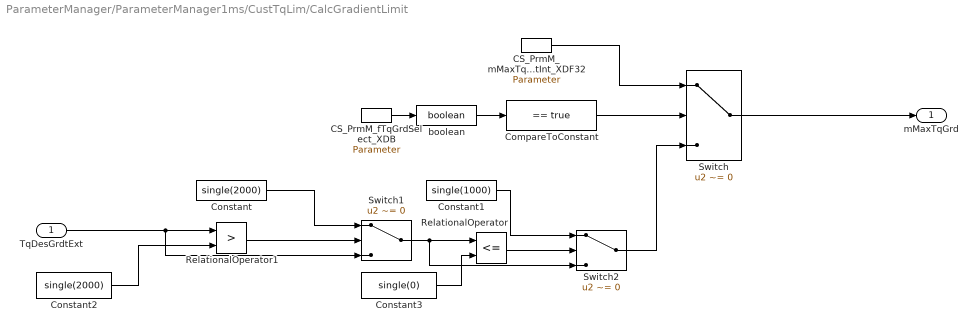
== system ParameterManager/ParameterManager1ms/CustTqLim/CalcGradientLimit ==
  TqDesGrdtExt : Inport
  CS_PrmM_fTqGrdSelect_XDB : CalibrationLib/Parameter  calParamName=CS_PrmM_fTqGrdSelect_XDB
      settings: AttributesFormatString=%<calParamName>  SourceProductName=SEG Calibration Lib
  CS_PrmM_mMaxTqGrdtInt_XDF32 : CalibrationLib/Parameter  calParamName=CS_PrmM_mMaxTqGrdtInt_XDF32
      settings: AttributesFormatString=%<calParamName>  SourceProductName=SEG Calibration Lib
  CompareToConstant : simulink/Logic and Bit Operations/Compare To Constant  relop===  const=true  OutDataTypeStr=boolean
  Constant : Constant  Value=single(2000)
  Constant1 : Constant  Value=single(1000)
  Constant2 : Constant  Value=single(2000)
  Constant3 : Constant  Value=single(0)
  RelationalOperator : RelationalOperator  Operator=<=  OutDataTypeStr=boolean  RndMeth=Simplest  InputSameDT=off
  RelationalOperator1 : RelationalOperator  Operator=>  OutDataTypeStr=boolean  RndMeth=Simplest  InputSameDT=off
  Switch : Switch  Criteria=u2 ~= 0  SaturateOnIntegerOverflow=off  InputSameDT=off
  Switch1 : Switch  Criteria=u2 ~= 0  SaturateOnIntegerOverflow=off  InputSameDT=off
  Switch2 : Switch  Criteria=u2 ~= 0  SaturateOnIntegerOverflow=off  InputSameDT=off
  boolean : DataTypeConversion  OutDataTypeStr=boolean  SaturateOnIntegerOverflow=off  RndMeth=Floor
  mMaxTqGrd : Outport  VectorParamsAs1DForOutWhenUnconnected=off
  wires:
  RelationalOperator/1 -> Switch2/2
  Constant/1 -> Switch1/1
  Constant1/1 -> Switch2/1
  TqDesGrdtExt/1 -> Switch1/3, RelationalOperator1/1
  Switch/1 -> mMaxTqGrd/1
  Switch2/1 -> Switch/3
  RelationalOperator1/1 -> Switch1/2
  Switch1/1 -> RelationalOperator/1, Switch2/3
  CS_PrmM_mMaxTqGrdtInt_XDF32/1 -> Switch/1
  Constant2/1 -> RelationalOperator1/2
  Constant3/1 -> RelationalOperator/2
  CS_PrmM_fTqGrdSelect_XDB/1 -> boolean/1
  boolean/1 -> CompareToConstant/1
  CompareToConstant/1 -> Switch/2

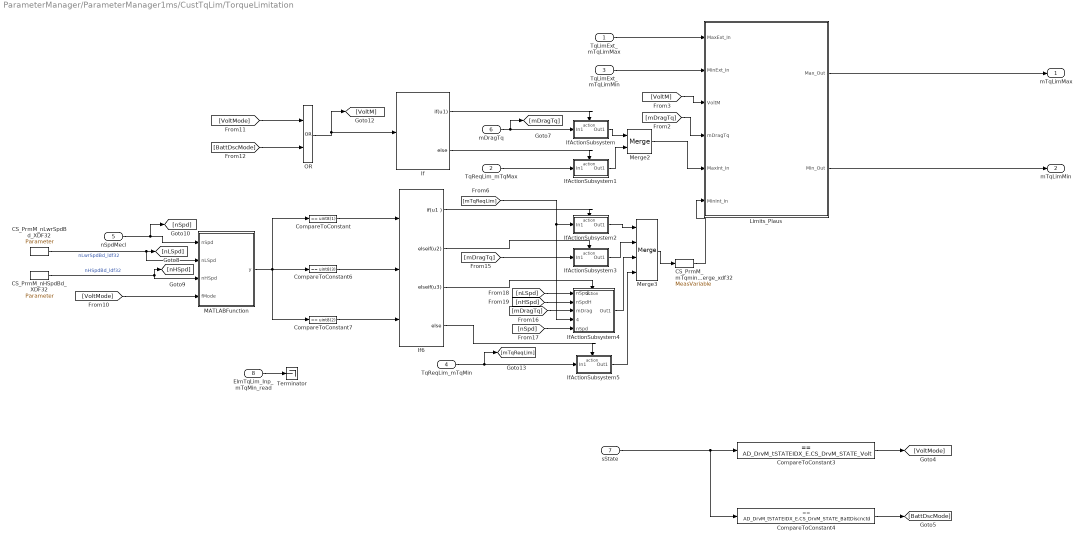
== system ParameterManager/ParameterManager1ms/CustTqLim/TorqueLimitation ==
  TqLimExt_mTqLimMax : Inport
  TqReqLim_mTqMax : Inport  Port=2
  TqLimExt_mTqLimMin : Inport  Port=3
  TqReqLim_mTqMin : Inport  Port=4
  nSpdMecl : Inport  Port=5
  mDragTq : Inport  Port=6
  sState : Inport  Port=7
  ElmTqLim_Inp_mTqMin_read : Inport  Port=8
  CS_PrmM_mTqminmerge_xdf32 : CalibrationLib/MeasVariable  calSigName=CS_PrmM_mTqminmerge_xdf32  logSignal=on
      settings: AttributesFormatString=%<calSigName>  SourceProductName=SEG Calibration Lib
  CS_PrmM_nHSpdBd_XDF32 : CalibrationLib/Parameter  calParamName=CS_PrmM_nHSpdBd_XDF32
      settings: AttributesFormatString=%<calParamName>  SourceProductName=SEG Calibration Lib
  CS_PrmM_nLwrSpdBd_XDF32 : CalibrationLib/Parameter  calParamName=CS_PrmM_nLwrSpdBd_XDF32
      settings: AttributesFormatString=%<calParamName>  SourceProductName=SEG Calibration Lib
  CompareToConstant : simulink/Logic and Bit Operations/Compare To Constant  relop===  const=uint8(1)  OutDataTypeStr=boolean
  CompareToConstant3 : simulink/Logic and Bit Operations/Compare To Constant  relop===  const=AD_DrvM_tSTATEIDX_E.CS_DrvM_STATE_Volt  OutDataTypeStr=boolean
  CompareToConstant4 : simulink/Logic and Bit Operations/Compare To Constant  relop===  const=AD_DrvM_tSTATEIDX_E.CS_DrvM_STATE_BattDiscnctd  OutDataTypeStr=boolean
  CompareToConstant6 : simulink/Logic and Bit Operations/Compare To Constant  relop===  const=uint8(3)  OutDataTypeStr=boolean
  CompareToConstant7 : simulink/Logic and Bit Operations/Compare To Constant  relop===  const=uint8(2)  OutDataTypeStr=boolean
  If : If  IfExpression=u1
  If6 : If  NumInputs=3  IfExpression=u1  ElseIfExpressions=u2,u3
  IfActionSubsystem : Subsystem  TreatAsAtomicUnit=on
  IfActionSubsystem1 : Subsystem  TreatAsAtomicUnit=on
  IfActionSubsystem2 : Subsystem  TreatAsAtomicUnit=on
  IfActionSubsystem3 : Subsystem  TreatAsAtomicUnit=on
  IfActionSubsystem4 : Subsystem  TreatAsAtomicUnit=on
  IfActionSubsystem5 : Subsystem  TreatAsAtomicUnit=on
  Limits_Plaus : Subsystem  AncestorBlock=ParameterManager/Limits_Plaus
  MATLABFunction : MATLAB Function  TreatAsAtomicUnit=on
  Merge2 : Merge
  Merge3 : Merge  Inputs=4
  OR : Logic  Operator=OR  AllPortsSameDT=off  OutDataTypeStr=boolean
  Terminator : Terminator
  mTqLimMax : Outport  VectorParamsAs1DForOutWhenUnconnected=off
  mTqLimMin : Outport  Port=2  VectorParamsAs1DForOutWhenUnconnected=off
  wires:
  [mDragTq] -> Limits_Plaus/4(mDragTq)
  nSpdMecl/1 -> [nSpd], MATLABFunction/1(nSpd)
  CompareToConstant/1 -> If6/1
  CS_PrmM_nHSpdBd_XDF32/1 -> MATLABFunction/3(nHSpd), [nHSpd]  "nHSpdBd_ldf32"
  CS_PrmM_nLwrSpdBd_XDF32/1 -> MATLABFunction/2(nLSpd), [nLSpd]  "nLwrSpdBd_ldf32"
  Merge2/1 -> Limits_Plaus/5(MaxInt_In)
  IfActionSubsystem1/1(Out1) -> Merge2/2
  TqReqLim_mTqMax/1 -> IfActionSubsystem1/1(In1)
  IfActionSubsystem/1(Out1) -> Merge2/1
  mDragTq/1 -> [mDragTq], IfActionSubsystem/1(In1)
  If/2 -> IfActionSubsystem1/Action
  If/1 -> IfActionSubsystem/Action
  OR/1 -> [VoltM], If/1
  [BattDscMode] -> OR/2
  [VoltMode] -> OR/1
  Limits_Plaus/1(Max_Out) -> mTqLimMax/1
  Limits_Plaus/2(Min_Out) -> mTqLimMin/1
  TqLimExt_mTqLimMin/1 -> Limits_Plaus/2(MinExt_In)
  TqLimExt_mTqLimMax/1 -> Limits_Plaus/1(MaxExt_In)
  sState/1 -> CompareToConstant4/1, CompareToConstant3/1
  [VoltMode] -> MATLABFunction/4(fMode)
  MATLABFunction/1(y) -> CompareToConstant/1, CompareToConstant6/1, CompareToConstant7/1
  If6/1 -> IfActionSubsystem2/Action
  ElmTqLim_Inp_mTqMin_read/1 -> Terminator/1
  IfActionSubsystem2/1(Out1) -> Merge3/1
  CompareToConstant6/1 -> If6/2
  CompareToConstant7/1 -> If6/3
  If6/2 -> IfActionSubsystem3/Action
  [mDragTq] -> IfActionSubsystem3/1(In1)
  IfActionSubsystem3/1(Out1) -> Merge3/2
  If6/3 -> IfActionSubsystem4/Action
  IfActionSubsystem4/1(Out1) -> Merge3/3
  If6/4 -> IfActionSubsystem5/Action
  TqReqLim_mTqMin/1 -> [mTqReqLim], IfActionSubsystem5/1(In1)
  IfActionSubsystem5/1(Out1) -> Merge3/4
  Merge3/1 -> CS_PrmM_mTqminmerge_xdf32/1
  CompareToConstant3/1 -> [VoltMode]
  CompareToConstant4/1 -> [BattDscMode]
  [VoltM] -> Limits_Plaus/3(VoltM)
  CS_PrmM_mTqminmerge_xdf32/1 -> Limits_Plaus/6(MinInt_In)
  [mDragTq] -> IfActionSubsystem4/3(mDrag)
  [nSpd] -> IfActionSubsystem4/5(nSpd)
  [nLSpd] -> IfActionSubsystem4/1(nSpdL)
  [nHSpd] -> IfActionSubsystem4/2(nSpdH)
  [mTqReqLim] -> IfActionSubsystem4/4(mTqMin), IfActionSubsystem2/1(In1)

== system ParameterManager/ParameterManager1ms/CustTqLim/TorqueLimitation/IfActionSubsystem ==
  In1 : Inport
  ActionPort : ActionPort
  Out1 : Outport  VectorParamsAs1DForOutWhenUnconnected=off
  wires:
  In1/1 -> Out1/1

== system ParameterManager/ParameterManager1ms/CustTqLim/TorqueLimitation/IfActionSubsystem1 ==
  In1 : Inport
  ActionPort : ActionPort
  Out1 : Outport  VectorParamsAs1DForOutWhenUnconnected=off
  wires:
  In1/1 -> Out1/1

== system ParameterManager/ParameterManager1ms/CustTqLim/TorqueLimitation/IfActionSubsystem2 ==
  In1 : Inport
  ActionPort : ActionPort
  Out1 : Outport  VectorParamsAs1DForOutWhenUnconnected=off
  wires:
  In1/1 -> Out1/1

== system ParameterManager/ParameterManager1ms/CustTqLim/TorqueLimitation/IfActionSubsystem3 ==
  In1 : Inport
  ActionPort : ActionPort
  Out1 : Outport  VectorParamsAs1DForOutWhenUnconnected=off
  wires:
  In1/1 -> Out1/1

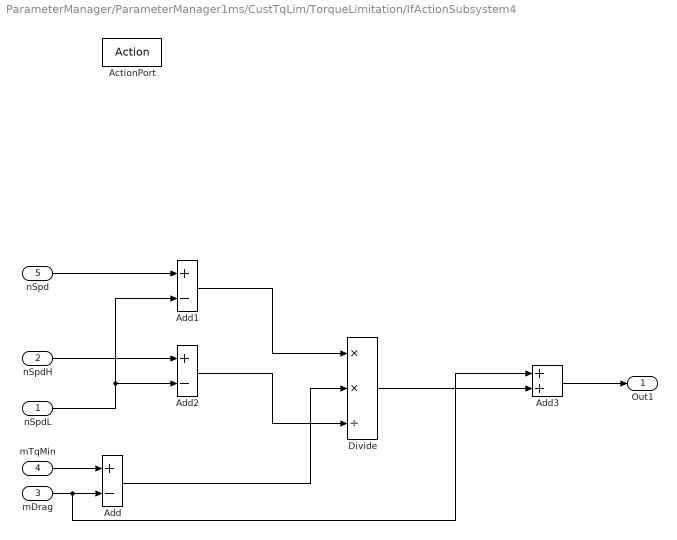
== system ParameterManager/ParameterManager1ms/CustTqLim/TorqueLimitation/IfActionSubsystem4 ==
  nSpdL : Inport
  nSpdH : Inport  Port=2
  mDrag : Inport  Port=3
  mTqMin : Inport  Port=4
  nSpd : Inport  Port=5
  ActionPort : ActionPort
  Add : Sum  Inputs=+-
  Add1 : Sum  Inputs=+-
  Add2 : Sum  Inputs=+-
  Add3 : Sum
  Divide : Product  Inputs=**/
  Out1 : Outport  VectorParamsAs1DForOutWhenUnconnected=off
  wires:
  mTqMin/1 -> Add/1
  mDrag/1 -> Add3/1, Add/2
  nSpd/1 -> Add1/1
  nSpdL/1 -> Add2/2, Add1/2
  nSpdH/1 -> Add2/1
  Add2/1 -> Divide/3
  Add1/1 -> Divide/1
  Add/1 -> Divide/2
  Divide/1 -> Add3/2
  Add3/1 -> Out1/1

== system ParameterManager/ParameterManager1ms/CustTqLim/TorqueLimitation/IfActionSubsystem5 ==
  In1 : Inport
  ActionPort : ActionPort
  Out1 : Outport  VectorParamsAs1DForOutWhenUnconnected=off
  wires:
  In1/1 -> Out1/1

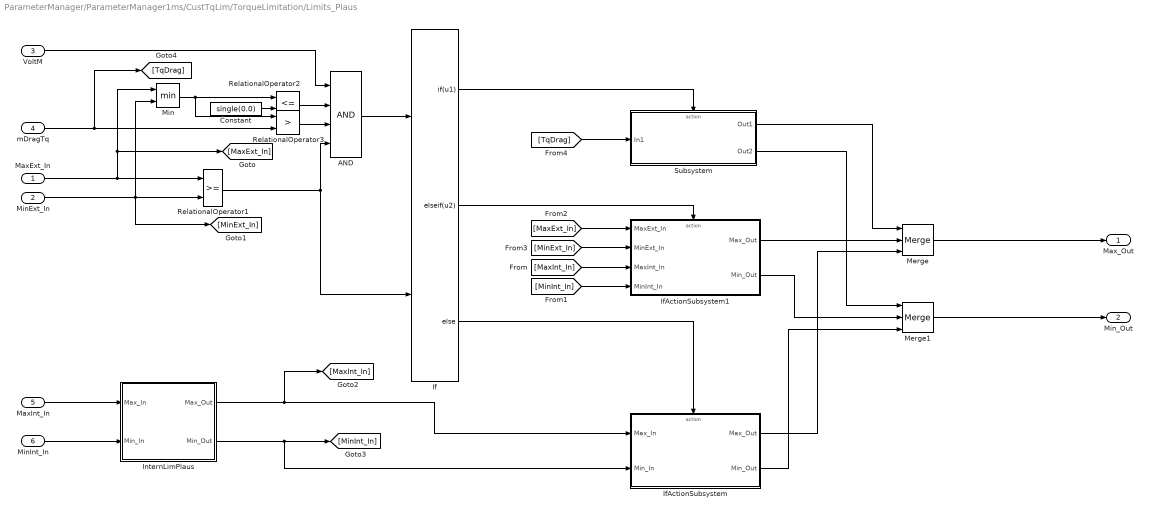
== system ParameterManager/ParameterManager1ms/CustTqLim/TorqueLimitation/Limits_Plaus ==
  MaxExt_In : Inport
  MinExt_In : Inport  Port=2
  VoltM : Inport  Port=3
  mDragTq : Inport  Port=4
  MaxInt_In : Inport  Port=5
  MinInt_In : Inport  Port=6
  AND : Logic  Inputs=4  AllPortsSameDT=off  OutDataTypeStr=boolean
  Constant : Constant  Value=single(0.0)
  If : If  NumInputs=2  IfExpression=u1  ElseIfExpressions=u2
  IfActionSubsystem : Subsystem  TreatAsAtomicUnit=on
  IfActionSubsystem1 : Subsystem  TreatAsAtomicUnit=on
  InternLimPlaus : Subsystem
  Merge : Merge  Inputs=3
  Merge1 : Merge  Inputs=3
  Min : MinMax  Inputs=2
  RelationalOperator1 : RelationalOperator  OutDataTypeStr=boolean  RndMeth=Simplest  InputSameDT=off
  RelationalOperator2 : RelationalOperator  Operator=<=  OutDataTypeStr=boolean  RndMeth=Simplest  InputSameDT=off
  RelationalOperator3 : RelationalOperator  Operator=>  OutDataTypeStr=boolean  RndMeth=Simplest  InputSameDT=off
  Subsystem : Subsystem
  Max_Out : Outport  VectorParamsAs1DForOutWhenUnconnected=off
  Min_Out : Outport  Port=2  VectorParamsAs1DForOutWhenUnconnected=off
  wires:
  MinInt_In/1 -> InternLimPlaus/2(Min_In)
  MaxInt_In/1 -> InternLimPlaus/1(Max_In)
  IfActionSubsystem/2(Min_Out) -> Merge1/3
  Merge1/1 -> Min_Out/1
  IfActionSubsystem1/1(Max_Out) -> Merge/2
  IfActionSubsystem/1(Max_Out) -> Merge/3
  IfActionSubsystem1/2(Min_Out) -> Merge1/2
  InternLimPlaus/1(Max_Out) -> IfActionSubsystem/1(Max_In), [MaxInt_In]
  If/3 -> IfActionSubsystem/Action
  [MinExt_In] -> IfActionSubsystem1/2(MinExt_In)
  [MaxExt_In] -> IfActionSubsystem1/1(MaxExt_In)
  Merge/1 -> Max_Out/1
  [MaxInt_In] -> IfActionSubsystem1/3(MaxInt_In)
  InternLimPlaus/2(Min_Out) -> [MinInt_In], IfActionSubsystem/2(Min_In)
  [MinInt_In] -> IfActionSubsystem1/4(MinInt_In)
  MaxExt_In/1 -> [MaxExt_In], Min/1, RelationalOperator1/1
  MinExt_In/1 -> Min/2, RelationalOperator1/2, [MinExt_In]
  Min/1 -> RelationalOperator3/1, RelationalOperator2/1
  mDragTq/1 -> [TqDrag], RelationalOperator3/2
  RelationalOperator2/1 -> AND/2
  RelationalOperator3/1 -> AND/3
  AND/1 -> If/1
  RelationalOperator1/1 -> If/2, AND/4
  If/2 -> IfActionSubsystem1/Action
  If/1 -> Subsystem/Action
  Subsystem/2(Out2) -> Merge1/1
  Subsystem/1(Out1) -> Merge/1
  Constant/1 -> RelationalOperator2/2
  [TqDrag] -> Subsystem/1(In1)
  VoltM/1 -> AND/1

== system ParameterManager/ParameterManager1ms/CustTqLim/TorqueLimitation/Limits_Plaus/IfActionSubsystem ==
  Max_In : Inport
  Min_In : Inport  Port=2
  ActionPort : ActionPort
  Max_Out : Outport  VectorParamsAs1DForOutWhenUnconnected=off
  Min_Out : Outport  Port=2  VectorParamsAs1DForOutWhenUnconnected=off
  wires:
  Min_In/1 -> Min_Out/1
  Max_In/1 -> Max_Out/1

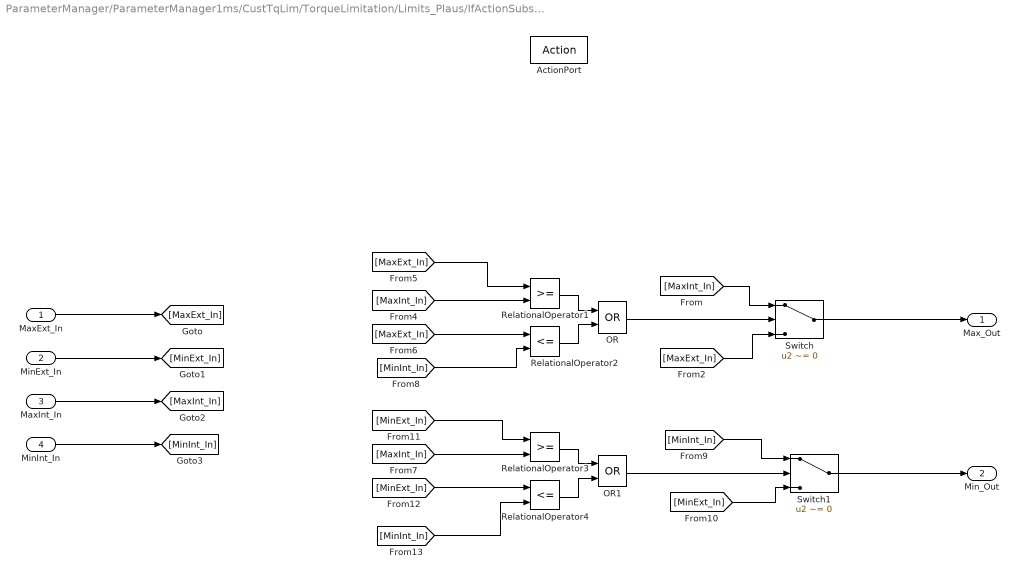
== system ParameterManager/ParameterManager1ms/CustTqLim/TorqueLimitation/Limits_Plaus/IfActionSubsystem1 ==
  MaxExt_In : Inport
  MinExt_In : Inport  Port=2
  MaxInt_In : Inport  Port=3
  MinInt_In : Inport  Port=4
  ActionPort : ActionPort
  OR : Logic  Operator=OR  AllPortsSameDT=off  OutDataTypeStr=boolean
  OR1 : Logic  Operator=OR  AllPortsSameDT=off  OutDataTypeStr=boolean
  RelationalOperator1 : RelationalOperator  OutDataTypeStr=boolean  RndMeth=Simplest  InputSameDT=off
  RelationalOperator2 : RelationalOperator  Operator=<=  OutDataTypeStr=boolean  RndMeth=Simplest  InputSameDT=off
  RelationalOperator3 : RelationalOperator  OutDataTypeStr=boolean  RndMeth=Simplest  InputSameDT=off
  RelationalOperator4 : RelationalOperator  Operator=<=  OutDataTypeStr=boolean  RndMeth=Simplest  InputSameDT=off
  Switch : Switch  Criteria=u2 ~= 0  SaturateOnIntegerOverflow=off  InputSameDT=off
  Switch1 : Switch  Criteria=u2 ~= 0  SaturateOnIntegerOverflow=off  InputSameDT=off
  Max_Out : Outport  VectorParamsAs1DForOutWhenUnconnected=off
  Min_Out : Outport  Port=2  VectorParamsAs1DForOutWhenUnconnected=off
  wires:
  [MinInt_In] -> RelationalOperator4/2
  [MinExt_In] -> RelationalOperator4/1
  [MinExt_In] -> RelationalOperator3/1
  [MinExt_In] -> Switch1/3
  [MinInt_In] -> Switch1/1
  [MinInt_In] -> RelationalOperator2/2
  [MaxInt_In] -> RelationalOperator3/2
  [MaxExt_In] -> RelationalOperator2/1
  [MaxExt_In] -> RelationalOperator1/1
  [MaxInt_In] -> RelationalOperator1/2
  [MaxInt_In] -> Switch/1
  [MaxExt_In] -> Switch/3
  MinExt_In/1 -> [MinExt_In]
  OR1/1 -> Switch1/2
  RelationalOperator3/1 -> OR1/1
  RelationalOperator4/1 -> OR1/2
  OR/1 -> Switch/2
  RelationalOperator2/1 -> OR/2
  RelationalOperator1/1 -> OR/1
  MinInt_In/1 -> [MinInt_In]
  MaxInt_In/1 -> [MaxInt_In]
  MaxExt_In/1 -> [MaxExt_In]
  Switch/1 -> Max_Out/1
  Switch1/1 -> Min_Out/1

== system ParameterManager/ParameterManager1ms/CustTqLim/TorqueLimitation/Limits_Plaus/InternLimPlaus ==
  Max_In : Inport
  Min_In : Inport  Port=2
  RelationalOperator1 : RelationalOperator  OutDataTypeStr=boolean  RndMeth=Simplest  InputSameDT=off
  Switch : Switch  Criteria=u2 ~= 0  SaturateOnIntegerOverflow=off  InputSameDT=off
  Switch1 : Switch  Criteria=u2 ~= 0  SaturateOnIntegerOverflow=off  InputSameDT=off
  Max_Out : Outport  VectorParamsAs1DForOutWhenUnconnected=off
  Min_Out : Outport  Port=2  VectorParamsAs1DForOutWhenUnconnected=off
  wires:
  Min_In/1 -> Switch1/1, Switch/3, RelationalOperator1/2
  Switch1/1 -> Min_Out/1
  Switch/1 -> Max_Out/1
  Max_In/1 -> RelationalOperator1/1, Switch/1, Switch1/3
  RelationalOperator1/1 -> Switch/2, Switch1/2

== system ParameterManager/ParameterManager1ms/CustTqLim/TorqueLimitation/Limits_Plaus/Subsystem ==
  In1 : Inport
  ActionPort : ActionPort
  Out1 : Outport  VectorParamsAs1DForOutWhenUnconnected=off
  Out2 : Outport  Port=2  VectorParamsAs1DForOutWhenUnconnected=off
  wires:
  In1/1 -> Out2/1, Out1/1

== matlab function ParameterManager/ParameterManager1ms/CustTqLim/TorqueLimitation/MATLABFunction ==
  data: nSpd input; y output; nLSpd input; nHSpd input; fMode input

function y = fcn(nSpd,nLSpd,nHSpd,fMode)
if fMode
    if nSpd>=nHSpd
        y=uint8(1);
    elseif nSpd>nLSpd
        y=uint8(2);
    else
        y=uint8(3);
    end
else
    y=uint8(0);
end
